simulink model "ASM_Traffic_new"  (R2024a)
settings: Solver=ode1  StartTime=SIM.tstart.v  StopTime=SIM.tend.v  FixedStep=SIM.StepSize.v  RelTol=1e-3
PostLoadFcn:
  | if any(exist('dsrtsu_mdlpostloadfcn', 'file') ~= 0), dsrtsu_mdlpostloadfcn('Execute', bdroot); end
  | try, asm_mdl_postloadfcn(bdroot, 'UpdateModel', 3600); catch, disp(lasterr); end,
InitFcn:
  | , if any(exist('rtifpga_mdlclblib', 'file') ~= 0), rtifpga_mdlclblib('Init', bdroot); end,
  | , if any(exist('dsmpb_private', 'file') ~= 0), dsmpb_private('dsmpb_mdlclblib', 'Init', bdroot); end,
undefined symbols (not defined in the file): _to_, a0b2, ASM_BrakeHydraulics_DemoSystems, ASM_VehicleDynamics_DemoSystems, b98103fe8ad365046cd0, BrakeCircuit, CPT, Crankshaft, DiscIntNeverNeededParam, dsmsi, FinalDriveAssembly, MDL, ModeSignals, Pos_BrakePedal_Maneuver, rad, RefSignals, s_to_rpm, SIM, SoftECU, Suspension, Tire, Transmission
libraries: ASM_Traffic_lib x135, simulink x100, ASM_Utils_lib x77, ASM_VehicleDynamics_lib x70, ASM_Environment_lib x22, dsmpblib x20, dsmsilib x15, MDLD_Utils_lib x10, ASM_BrakeHydraulics_lib x3
(part 24 of 63)

== system ASM_Traffic_new/Environment/Interface_Out/Animation/Mnv_Trunk[]_ ==
  In1 : Inport
  Gain : Gain  SaturateOnIntegerOverflow=on  OutDataTypeStr=Inherit: Same as input  ParamDataTypeStr=Inherit: Same as input
  Out1 : Outport  VectorParamsAs1DForOutWhenUnconnected=off
  wires:
  Gain/1 -> Out1/1
  In1/1 -> Gain/1

== system ASM_Traffic_new/Environment/Interface_Out/Animation/Network_Item_Type_Veh[]_ ==
  In1 : Inport
  Gain : Gain  SaturateOnIntegerOverflow=on  OutDataTypeStr=Inherit: Same as input  ParamDataTypeStr=Inherit: Same as input
  Out1 : Outport  VectorParamsAs1DForOutWhenUnconnected=off
  wires:
  Gain/1 -> Out1/1
  In1/1 -> Gain/1

== system ASM_Traffic_new/Environment/Interface_Out/Animation/Pos_Left[x;y;z][m]_ ==
  In1 : Inport
  Gain : Gain  SaturateOnIntegerOverflow=on  OutDataTypeStr=Inherit: Same as input  ParamDataTypeStr=Inherit: Same as input
  Out1 : Outport  VectorParamsAs1DForOutWhenUnconnected=off
  wires:
  Gain/1 -> Out1/1
  In1/1 -> Gain/1

== system ASM_Traffic_new/Environment/Interface_Out/Animation/Pos_Right[x;y;z][m]_ ==
  In1 : Inport
  Gain : Gain  SaturateOnIntegerOverflow=on  OutDataTypeStr=Inherit: Same as input  ParamDataTypeStr=Inherit: Same as input
  Out1 : Outport  VectorParamsAs1DForOutWhenUnconnected=off
  wires:
  In1/1 -> Gain/1
  Gain/1 -> Out1/1

== system ASM_Traffic_new/Environment/Interface_Out/Animation/Sw_AnimationInterface[0Disabled|1Enabled]_ ==
  In1 : Inport
  Gain : Gain  SaturateOnIntegerOverflow=on  OutDataTypeStr=Inherit: Same as input  ParamDataTypeStr=Inherit: Same as input
  Out1 : Outport  VectorParamsAs1DForOutWhenUnconnected=off
  wires:
  Gain/1 -> Out1/1
  In1/1 -> Gain/1

== system ASM_Traffic_new/Environment/Interface_Out/Animation/Sw_BrakeLight[0Off|1On]_ ==
  In1 : Inport
  Gain : Gain  SaturateOnIntegerOverflow=on  OutDataTypeStr=Inherit: Same as input  ParamDataTypeStr=Inherit: Same as input
  Out1 : Outport  VectorParamsAs1DForOutWhenUnconnected=off
  wires:
  Gain/1 -> Out1/1
  In1/1 -> Gain/1

== system ASM_Traffic_new/Environment/Interface_Out/Animation/Sw_DoorFL[0Closed_1Open]_ ==
  In1 : Inport
  Gain : Gain  SaturateOnIntegerOverflow=on  OutDataTypeStr=Inherit: Same as input  ParamDataTypeStr=Inherit: Same as input
  Out1 : Outport  VectorParamsAs1DForOutWhenUnconnected=off
  wires:
  Gain/1 -> Out1/1
  In1/1 -> Gain/1

== system ASM_Traffic_new/Environment/Interface_Out/Animation/Sw_DoorFR[0Closed_1Open]_ ==
  In1 : Inport
  Gain : Gain  SaturateOnIntegerOverflow=on  OutDataTypeStr=Inherit: Same as input  ParamDataTypeStr=Inherit: Same as input
  Out1 : Outport  VectorParamsAs1DForOutWhenUnconnected=off
  wires:
  Gain/1 -> Out1/1
  In1/1 -> Gain/1

== system ASM_Traffic_new/Environment/Interface_Out/Animation/Sw_DoorRL[0Closed_1Open]_ ==
  In1 : Inport
  Gain : Gain  SaturateOnIntegerOverflow=on  OutDataTypeStr=Inherit: Same as input  ParamDataTypeStr=Inherit: Same as input
  Out1 : Outport  VectorParamsAs1DForOutWhenUnconnected=off
  wires:
  Gain/1 -> Out1/1
  In1/1 -> Gain/1

== system ASM_Traffic_new/Environment/Interface_Out/Animation/Sw_DoorRR[0Closed_1Open]_ ==
  In1 : Inport
  Gain : Gain  SaturateOnIntegerOverflow=on  OutDataTypeStr=Inherit: Same as input  ParamDataTypeStr=Inherit: Same as input
  Out1 : Outport  VectorParamsAs1DForOutWhenUnconnected=off
  wires:
  In1/1 -> Gain/1
  Gain/1 -> Out1/1

== system ASM_Traffic_new/Environment/Interface_Out/Animation/Sw_Hood[0Closed_1Open]_ ==
  In1 : Inport
  Gain : Gain  SaturateOnIntegerOverflow=on  OutDataTypeStr=Inherit: Same as input  ParamDataTypeStr=Inherit: Same as input
  Out1 : Outport  VectorParamsAs1DForOutWhenUnconnected=off
  wires:
  Gain/1 -> Out1/1
  In1/1 -> Gain/1

== system ASM_Traffic_new/Environment/Interface_Out/Animation/Sw_ManualControl_Doors[1Maneuver|2Manual]_ ==
  In1 : Inport
  Gain : Gain  SaturateOnIntegerOverflow=on  OutDataTypeStr=Inherit: Same as input  ParamDataTypeStr=Inherit: Same as input
  Out1 : Outport  VectorParamsAs1DForOutWhenUnconnected=off
  wires:
  Gain/1 -> Out1/1
  In1/1 -> Gain/1

== system ASM_Traffic_new/Environment/Interface_Out/Animation/Sw_ManualControl_Lights[1Maneuver|2Manual]_ ==
  In1 : Inport
  Gain : Gain  SaturateOnIntegerOverflow=on  OutDataTypeStr=Inherit: Same as input  ParamDataTypeStr=Inherit: Same as input
  Out1 : Outport  VectorParamsAs1DForOutWhenUnconnected=off
  wires:
  In1/1 -> Gain/1
  Gain/1 -> Out1/1

== system ASM_Traffic_new/Environment/Interface_Out/Animation/Sw_Trunk[0Closed_1Open]_ ==
  In1 : Inport
  Gain : Gain  SaturateOnIntegerOverflow=on  OutDataTypeStr=Inherit: Same as input  ParamDataTypeStr=Inherit: Same as input
  Out1 : Outport  VectorParamsAs1DForOutWhenUnconnected=off
  wires:
  In1/1 -> Gain/1
  Gain/1 -> Out1/1

== system ASM_Traffic_new/Environment/Interface_Out/Animation/Sw_TurnLights[0Off|1Left|2Right|3Both]_ ==
  In1 : Inport
  Gain : Gain  SaturateOnIntegerOverflow=on  OutDataTypeStr=Inherit: Same as input  ParamDataTypeStr=Inherit: Same as input
  Out1 : Outport  VectorParamsAs1DForOutWhenUnconnected=off
  wires:
  In1/1 -> Gain/1
  Gain/1 -> Out1/1

== system ASM_Traffic_new/Environment/Interface_Out/Animation/Velocity_MeasPnt_Marker_Left[m|s]_ ==
  In1 : Inport
  Gain : Gain  SaturateOnIntegerOverflow=on  OutDataTypeStr=Inherit: Same as input  ParamDataTypeStr=Inherit: Same as input
  Out1 : Outport  VectorParamsAs1DForOutWhenUnconnected=off
  wires:
  In1/1 -> Gain/1
  Gain/1 -> Out1/1

== system ASM_Traffic_new/Environment/Interface_Out/Animation/Velocity_MeasPnt_Marker_Right[m|s]_ ==
  In1 : Inport
  Gain : Gain  SaturateOnIntegerOverflow=on  OutDataTypeStr=Inherit: Same as input  ParamDataTypeStr=Inherit: Same as input
  Out1 : Outport  VectorParamsAs1DForOutWhenUnconnected=off
  wires:
  Gain/1 -> Out1/1
  In1/1 -> Gain/1

== system ASM_Traffic_new/Environment/Interface_Out/Animation/Yaw_Angle_Left[deg]_ ==
  In1 : Inport
  Gain : Gain  SaturateOnIntegerOverflow=on  OutDataTypeStr=Inherit: Same as input  ParamDataTypeStr=Inherit: Same as input
  Out1 : Outport  VectorParamsAs1DForOutWhenUnconnected=off
  wires:
  In1/1 -> Gain/1
  Gain/1 -> Out1/1

== system ASM_Traffic_new/Environment/Interface_Out/Animation/Yaw_Angle_Right[deg]_ ==
  In1 : Inport
  Gain : Gain  SaturateOnIntegerOverflow=on  OutDataTypeStr=Inherit: Same as input  ParamDataTypeStr=Inherit: Same as input
  Out1 : Outport  VectorParamsAs1DForOutWhenUnconnected=off
  wires:
  Gain/1 -> Out1/1
  In1/1 -> Gain/1

== system ASM_Traffic_new/Environment/Interface_Out/Animation/a_Fellows[m|s2] ==
  In1 : Inport
  Gain : Gain  SaturateOnIntegerOverflow=on  OutDataTypeStr=Inherit: Same as input  ParamDataTypeStr=Inherit: Same as input
  Out1 : Outport  VectorParamsAs1DForOutWhenUnconnected=off
  wires:
  Gain/1 -> Out1/1
  In1/1 -> Gain/1

== system ASM_Traffic_new/Environment/Interface_Out/Animation/s_Veh_Road[m]_ ==
  In1 : Inport
  Gain : Gain  SaturateOnIntegerOverflow=on  OutDataTypeStr=Inherit: Same as input  ParamDataTypeStr=Inherit: Same as input
  Out1 : Outport  VectorParamsAs1DForOutWhenUnconnected=off
  wires:
  In1/1 -> Gain/1
  Gain/1 -> Out1/1

== system ASM_Traffic_new/Environment/Interface_Out/Animation/v_Fellows[km|h]_ ==
  In1 : Inport
  Gain : Gain  SaturateOnIntegerOverflow=on  OutDataTypeStr=Inherit: Same as input  ParamDataTypeStr=Inherit: Same as input
  Out1 : Outport  VectorParamsAs1DForOutWhenUnconnected=off
  wires:
  In1/1 -> Gain/1
  Gain/1 -> Out1/1

== system ASM_Traffic_new/Environment/Interface_Out/Animation/v_Fellows_Ref_Scheduler[km|h]_ ==
  In1 : Inport
  Gain : Gain  SaturateOnIntegerOverflow=on  OutDataTypeStr=Inherit: Same as input  ParamDataTypeStr=Inherit: Same as input
  Out1 : Outport  VectorParamsAs1DForOutWhenUnconnected=off
  wires:
  Gain/1 -> Out1/1
  In1/1 -> Gain/1

== system ASM_Traffic_new/Environment/Interface_Out/Plant_ModelSignals/Activate_DCLink[0Off|1On]_ ==
  In1 : Inport
  Gain : Gain  SaturateOnIntegerOverflow=on  OutDataTypeStr=Inherit: Same as input  ParamDataTypeStr=Inherit: Same as input
  Out1 : Outport  VectorParamsAs1DForOutWhenUnconnected=off
  wires:
  In1/1 -> Gain/1
  Gain/1 -> Out1/1

== system ASM_Traffic_new/Environment/Interface_Out/Plant_ModelSignals/Angle_Hor_Rel_Fellows[deg]_ ==
  In1 : Inport
  Gain : Gain  SaturateOnIntegerOverflow=on  OutDataTypeStr=Inherit: Same as input  ParamDataTypeStr=Inherit: Same as input
  Out1 : Outport  VectorParamsAs1DForOutWhenUnconnected=off
  wires:
  In1/1 -> Gain/1
  Gain/1 -> Out1/1

== system ASM_Traffic_new/Environment/Interface_Out/Plant_ModelSignals/Angle_SteeringWheel_Maneuver[deg]_ ==
  In1 : Inport
  DummyGain : Gain  SaturateOnIntegerOverflow=on  OutDataTypeStr=Inherit: Same as input  ParamDataTypeStr=Inherit: Same as input
  Out1 : Outport  VectorParamsAs1DForOutWhenUnconnected=off
  wires:
  DummyGain/1 -> Out1/1
  In1/1 -> DummyGain/1

== system ASM_Traffic_new/Environment/Interface_Out/Plant_ModelSignals/Angle_Vehicle_Init_CoorSys_E[x;y;z][rad]_ ==
  In1 : Inport
  Gain : Gain  SaturateOnIntegerOverflow=on  OutDataTypeStr=Inherit: Same as input  ParamDataTypeStr=Inherit: Same as input
  Out1 : Outport  VectorParamsAs1DForOutWhenUnconnected=off
  wires:
  In1/1 -> Gain/1
  Gain/1 -> Out1/1

== system ASM_Traffic_new/Environment/Interface_Out/Plant_ModelSignals/Angle_Yaw_Veh_Road[deg]_ ==
  In1 : Inport
  Gain : Gain  SaturateOnIntegerOverflow=on  OutDataTypeStr=Inherit: Same as input  ParamDataTypeStr=Inherit: Same as input
  Out1 : Outport  VectorParamsAs1DForOutWhenUnconnected=off
  wires:
  In1/1 -> Gain/1
  Gain/1 -> Out1/1

== system ASM_Traffic_new/Environment/Interface_Out/Plant_ModelSignals/Const_Steering_Mode_Manual[1Angle|2Trq]_ ==
  In1 : Inport
  Gain : Gain  SaturateOnIntegerOverflow=on  OutDataTypeStr=Inherit: Same as input  ParamDataTypeStr=Inherit: Same as input
  Out1 : Outport  VectorParamsAs1DForOutWhenUnconnected=off
  wires:
  In1/1 -> Gain/1
  Gain/1 -> Out1/1

== system ASM_Traffic_new/Environment/Interface_Out/Plant_ModelSignals/Curv_Preview_Road[1|m]_ ==
  In1 : Inport
  Gain : Gain  SaturateOnIntegerOverflow=on  OutDataTypeStr=Inherit: Same as input  ParamDataTypeStr=Inherit: Same as input
  Out1 : Outport  VectorParamsAs1DForOutWhenUnconnected=off
  wires:
  Gain/1 -> Out1/1
  In1/1 -> Gain/1

== system ASM_Traffic_new/Environment/Interface_Out/Plant_ModelSignals/Curv_Vehicle_Road[1|m]_ ==
  In1 : Inport
  Gain : Gain  SaturateOnIntegerOverflow=on  OutDataTypeStr=Inherit: Same as input  ParamDataTypeStr=Inherit: Same as input
  Out1 : Outport  VectorParamsAs1DForOutWhenUnconnected=off
  wires:
  Gain/1 -> Out1/1
  In1/1 -> Gain/1

== system ASM_Traffic_new/Environment/Interface_Out/Plant_ModelSignals/Dist_Border_Left[m]_ ==
  In1 : Inport
  Gain : Gain  SaturateOnIntegerOverflow=on  OutDataTypeStr=Inherit: Same as input  ParamDataTypeStr=Inherit: Same as input
  Out1 : Outport  VectorParamsAs1DForOutWhenUnconnected=off
  wires:
  Gain/1 -> Out1/1
  In1/1 -> Gain/1

== system ASM_Traffic_new/Environment/Interface_Out/Plant_ModelSignals/Dist_Border_Right[m]_ ==
  In1 : Inport
  Gain : Gain  SaturateOnIntegerOverflow=on  OutDataTypeStr=Inherit: Same as input  ParamDataTypeStr=Inherit: Same as input
  Out1 : Outport  VectorParamsAs1DForOutWhenUnconnected=off
  wires:
  In1/1 -> Gain/1
  Gain/1 -> Out1/1

== system ASM_Traffic_new/Environment/Interface_Out/Plant_ModelSignals/Dist_Fellows[m]_ ==
  In1 : Inport
  Gain : Gain  SaturateOnIntegerOverflow=on  OutDataTypeStr=Inherit: Same as input  ParamDataTypeStr=Inherit: Same as input
  Out1 : Outport  VectorParamsAs1DForOutWhenUnconnected=off
  wires:
  In1/1 -> Gain/1
  Gain/1 -> Out1/1

== system ASM_Traffic_new/Environment/Interface_Out/Plant_ModelSignals/ECU_Commands[]_ ==
  In1 : Inport
  Gain : Gain  SaturateOnIntegerOverflow=on  OutDataTypeStr=Inherit: Same as input  ParamDataTypeStr=Inherit: Same as input
  Out1 : Outport  VectorParamsAs1DForOutWhenUnconnected=off
  wires:
  In1/1 -> Gain/1
  Gain/1 -> Out1/1

== system ASM_Traffic_new/Environment/Interface_Out/Plant_ModelSignals/Enable_v_Init[0|1]_ ==
  In1 : Inport
  DummyGain : Gain  SaturateOnIntegerOverflow=on  OutDataTypeStr=Inherit: Same as input  ParamDataTypeStr=Inherit: Same as input
  Out1 : Outport  VectorParamsAs1DForOutWhenUnconnected=off
  wires:
  DummyGain/1 -> Out1/1
  In1/1 -> DummyGain/1

== system ASM_Traffic_new/Environment/Interface_Out/Plant_ModelSignals/EngOPNum[]_ ==
  In1 : Inport
  DummyGain : Gain  SaturateOnIntegerOverflow=on  OutDataTypeStr=Inherit: Same as input  ParamDataTypeStr=Inherit: Same as input
  Out1 : Outport  VectorParamsAs1DForOutWhenUnconnected=off
  wires:
  DummyGain/1 -> Out1/1
  In1/1 -> DummyGain/1

== system ASM_Traffic_new/Environment/Interface_Out/Plant_ModelSignals/Fric_Coeff_CP[:][]_ ==
  In1 : Inport
  Gain : Gain  SaturateOnIntegerOverflow=on  OutDataTypeStr=Inherit: Same as input  ParamDataTypeStr=Inherit: Same as input
  Out1 : Outport  VectorParamsAs1DForOutWhenUnconnected=off
  wires:
  In1/1 -> Gain/1
  Gain/1 -> Out1/1

== system ASM_Traffic_new/Environment/Interface_Out/Plant_ModelSignals/Gear_Maneuver[]_ ==
  In1 : Inport
  DummyGain : Gain  SaturateOnIntegerOverflow=on  OutDataTypeStr=Inherit: Same as input  ParamDataTypeStr=Inherit: Same as input
  Out1 : Outport  VectorParamsAs1DForOutWhenUnconnected=off
  wires:
  In1/1 -> DummyGain/1
  DummyGain/1 -> Out1/1

== system ASM_Traffic_new/Environment/Interface_Out/Plant_ModelSignals/Gear_Max[0Off|1_n]_ ==
  In1 : Inport
  DummyGain : Gain  SaturateOnIntegerOverflow=on  OutDataTypeStr=Inherit: Same as input  ParamDataTypeStr=Inherit: Same as input
  Out1 : Outport  VectorParamsAs1DForOutWhenUnconnected=off
  wires:
  In1/1 -> DummyGain/1
  DummyGain/1 -> Out1/1

== system ASM_Traffic_new/Environment/Interface_Out/Plant_ModelSignals/Height_Fellows[m]_ ==
  In1 : Inport
  Gain : Gain  SaturateOnIntegerOverflow=on  OutDataTypeStr=Inherit: Same as input  ParamDataTypeStr=Inherit: Same as input
  Out1 : Outport  VectorParamsAs1DForOutWhenUnconnected=off
  wires:
  In1/1 -> Gain/1
  Gain/1 -> Out1/1

== system ASM_Traffic_new/Environment/Interface_Out/Plant_ModelSignals/I_Load_HV[A]_ ==
  In1 : Inport
  Gain : Gain  SaturateOnIntegerOverflow=on  OutDataTypeStr=Inherit: Same as input  ParamDataTypeStr=Inherit: Same as input
  Out1 : Outport  VectorParamsAs1DForOutWhenUnconnected=off
  wires:
  Gain/1 -> Out1/1
  In1/1 -> Gain/1

== system ASM_Traffic_new/Environment/Interface_Out/Plant_ModelSignals/I_Load_LV[A]_ ==
  In1 : Inport
  Gain : Gain  SaturateOnIntegerOverflow=on  OutDataTypeStr=Inherit: Same as input  ParamDataTypeStr=Inherit: Same as input
  Out1 : Outport  VectorParamsAs1DForOutWhenUnconnected=off
  wires:
  In1/1 -> Gain/1
  Gain/1 -> Out1/1

== system ASM_Traffic_new/Environment/Interface_Out/Plant_ModelSignals/Keep_VehiclePosition[0|1]_ ==
  In1 : Inport
  Gain : Gain  SaturateOnIntegerOverflow=on  OutDataTypeStr=Inherit: Same as input  ParamDataTypeStr=Inherit: Same as input
  Out1 : Outport  VectorParamsAs1DForOutWhenUnconnected=off
  wires:
  In1/1 -> Gain/1
  Gain/1 -> Out1/1

== system ASM_Traffic_new/Environment/Interface_Out/Plant_ModelSignals/Lane_ID_Vehicle[]_ ==
  In1 : Inport
  Gain : Gain  SaturateOnIntegerOverflow=on  OutDataTypeStr=Inherit: Same as input  ParamDataTypeStr=Inherit: Same as input
  Out1 : Outport  VectorParamsAs1DForOutWhenUnconnected=off
  wires:
  In1/1 -> Gain/1
  Gain/1 -> Out1/1

== system ASM_Traffic_new/Environment/Interface_Out/Plant_ModelSignals/Length_Fellows[m]_ ==
  In1 : Inport
  Gain : Gain  SaturateOnIntegerOverflow=on  OutDataTypeStr=Inherit: Same as input  ParamDataTypeStr=Inherit: Same as input
  Out1 : Outport  VectorParamsAs1DForOutWhenUnconnected=off
  wires:
  In1/1 -> Gain/1
  Gain/1 -> Out1/1

== system ASM_Traffic_new/Environment/Interface_Out/Plant_ModelSignals/Mode_AcceleratorBrake[1Stim|2Driver]_ ==
  In1 : Inport
  Gain : Gain  SaturateOnIntegerOverflow=on  OutDataTypeStr=Inherit: Same as input  ParamDataTypeStr=Inherit: Same as input
  Out1 : Outport  VectorParamsAs1DForOutWhenUnconnected=off
  wires:
  In1/1 -> Gain/1
  Gain/1 -> Out1/1

== system ASM_Traffic_new/Environment/Interface_Out/Plant_ModelSignals/Mode_AdaptVelocityToRoad[1Off|2On]_ ==
  In1 : Inport
  Gain : Gain  SaturateOnIntegerOverflow=on  OutDataTypeStr=Inherit: Same as input  ParamDataTypeStr=Inherit: Same as input
  Out1 : Outport  VectorParamsAs1DForOutWhenUnconnected=off
  wires:
  In1/1 -> Gain/1
  Gain/1 -> Out1/1

== system ASM_Traffic_new/Environment/Interface_Out/Plant_ModelSignals/Mode_CurvatureCalculation[1Road|2Driver]_ ==
  In1 : Inport
  Gain : Gain  SaturateOnIntegerOverflow=on  OutDataTypeStr=Inherit: Same as input  ParamDataTypeStr=Inherit: Same as input
  Out1 : Outport  VectorParamsAs1DForOutWhenUnconnected=off
  wires:
  In1/1 -> Gain/1
  Gain/1 -> Out1/1

== system ASM_Traffic_new/Environment/Interface_Out/Plant_ModelSignals/Mode_ForceToRoad[1Off|2On]_ ==
  In1 : Inport
  Gain : Gain  SaturateOnIntegerOverflow=on  OutDataTypeStr=Inherit: Same as input  ParamDataTypeStr=Inherit: Same as input
  Out1 : Outport  VectorParamsAs1DForOutWhenUnconnected=off
  wires:
  Gain/1 -> Out1/1
  In1/1 -> Gain/1

== system ASM_Traffic_new/Environment/Interface_Out/Plant_ModelSignals/Mode_GearClutch[1Stim|2Driver|3OpenClutch|4RefGear]_ ==
  In1 : Inport
  Gain : Gain  SaturateOnIntegerOverflow=on  OutDataTypeStr=Inherit: Same as input  ParamDataTypeStr=Inherit: Same as input
  Out1 : Outport  VectorParamsAs1DForOutWhenUnconnected=off
  wires:
  Gain/1 -> Out1/1
  In1/1 -> Gain/1

== system ASM_Traffic_new/Environment/Interface_Out/Plant_ModelSignals/Mode_LatCtrl[1Pos|2Yaw]_ ==
  In1 : Inport
  Gain : Gain  SaturateOnIntegerOverflow=on  OutDataTypeStr=Inherit: Same as input  ParamDataTypeStr=Inherit: Same as input
  Out1 : Outport  VectorParamsAs1DForOutWhenUnconnected=off
  wires:
  Gain/1 -> Out1/1
  In1/1 -> Gain/1

== system ASM_Traffic_new/Environment/Interface_Out/Plant_ModelSignals/Mode_RelativeLane[0CenterLane|1PreferredLane]_ ==
  In1 : Inport
  Gain : Gain  SaturateOnIntegerOverflow=on  OutDataTypeStr=Inherit: Same as input  ParamDataTypeStr=Inherit: Same as input
  Out1 : Outport  VectorParamsAs1DForOutWhenUnconnected=off
  wires:
  In1/1 -> Gain/1
  Gain/1 -> Out1/1

== system ASM_Traffic_new/Environment/Interface_Out/Plant_ModelSignals/Mode_Road[1NoRoad|2Straight|3Circle|4Road]_ ==
  In1 : Inport
  Gain : Gain  SaturateOnIntegerOverflow=on  OutDataTypeStr=Inherit: Same as input  ParamDataTypeStr=Inherit: Same as input
  Out1 : Outport  VectorParamsAs1DForOutWhenUnconnected=off
  wires:
  Gain/1 -> Out1/1
  In1/1 -> Gain/1

== system ASM_Traffic_new/Environment/Interface_Out/Plant_ModelSignals/Mode_SelectorLever[1Stim|2Driver]_ ==
  In1 : Inport
  Gain : Gain  SaturateOnIntegerOverflow=on  OutDataTypeStr=Inherit: Same as input  ParamDataTypeStr=Inherit: Same as input
  Out1 : Outport  VectorParamsAs1DForOutWhenUnconnected=off
  wires:
  In1/1 -> Gain/1
  Gain/1 -> Out1/1

== system ASM_Traffic_new/Environment/Interface_Out/Plant_ModelSignals/Mode_StartButtonState[1Stim|2SoftECU]_ ==
  In1 : Inport
  Gain : Gain  SaturateOnIntegerOverflow=on  OutDataTypeStr=Inherit: Same as input  ParamDataTypeStr=Inherit: Same as input
  Out1 : Outport  VectorParamsAs1DForOutWhenUnconnected=off
  wires:
  Gain/1 -> Out1/1
  In1/1 -> Gain/1

== system ASM_Traffic_new/Environment/Interface_Out/Plant_ModelSignals/Mode_Steer[1Stim|2Driver|3Fix]_ ==
  In1 : Inport
  Gain : Gain  SaturateOnIntegerOverflow=on  OutDataTypeStr=Inherit: Same as input  ParamDataTypeStr=Inherit: Same as input
  Out1 : Outport  VectorParamsAs1DForOutWhenUnconnected=off
  wires:
  In1/1 -> Gain/1
  Gain/1 -> Out1/1

== system ASM_Traffic_new/Environment/Interface_Out/Plant_ModelSignals/Mode_TrafficDriver[1Off|2On]_ ==
  In1 : Inport
  Gain : Gain  SaturateOnIntegerOverflow=on  OutDataTypeStr=Inherit: Same as input  ParamDataTypeStr=Inherit: Same as input
  Out1 : Outport  VectorParamsAs1DForOutWhenUnconnected=off
  wires:
  Gain/1 -> Out1/1
  In1/1 -> Gain/1

== system ASM_Traffic_new/Environment/Interface_Out/Plant_ModelSignals/Object_ID[]_ ==
  In1 : Inport
  Gain : Gain  SaturateOnIntegerOverflow=on  OutDataTypeStr=Inherit: Same as input  ParamDataTypeStr=Inherit: Same as input
  Out1 : Outport  VectorParamsAs1DForOutWhenUnconnected=off
  wires:
  In1/1 -> Gain/1
  Gain/1 -> Out1/1

== system ASM_Traffic_new/Environment/Interface_Out/Plant_ModelSignals/Pitch_Preview_Road[deg]_ ==
  In1 : Inport
  Gain : Gain  SaturateOnIntegerOverflow=on  OutDataTypeStr=Inherit: Same as input  ParamDataTypeStr=Inherit: Same as input
  Out1 : Outport  VectorParamsAs1DForOutWhenUnconnected=off
  wires:
  Gain/1 -> Out1/1
  In1/1 -> Gain/1

== system ASM_Traffic_new/Environment/Interface_Out/Plant_ModelSignals/PosVec_MainPnt_Fellows[x;y;z][m]_ ==
  In1 : Inport
  Gain : Gain  SaturateOnIntegerOverflow=on  OutDataTypeStr=Inherit: Same as input  ParamDataTypeStr=Inherit: Same as input
  Out1 : Outport  VectorParamsAs1DForOutWhenUnconnected=off
  wires:
  In1/1 -> Gain/1
  Gain/1 -> Out1/1

== system ASM_Traffic_new/Environment/Interface_Out/Plant_ModelSignals/Pos_AccPedal_Maneuver[%]_ ==
  In1 : Inport
  DummyGain : Gain  SaturateOnIntegerOverflow=on  OutDataTypeStr=Inherit: Same as input  ParamDataTypeStr=Inherit: Same as input
  Out1 : Outport  VectorParamsAs1DForOutWhenUnconnected=off
  wires:
  In1/1 -> DummyGain/1
  DummyGain/1 -> Out1/1

== system ASM_Traffic_new/Environment/Interface_Out/Plant_ModelSignals/Pos_BrakePedal_Maneuver[%]_ ==
  In1 : Inport
  DummyGain : Gain  SaturateOnIntegerOverflow=on  OutDataTypeStr=Inherit: Same as input  ParamDataTypeStr=Inherit: Same as input
  Out1 : Outport  VectorParamsAs1DForOutWhenUnconnected=off
  wires:
  In1/1 -> DummyGain/1
  DummyGain/1 -> Out1/1

== system ASM_Traffic_new/Environment/Interface_Out/Plant_ModelSignals/Pos_ClutchPedal_Maneuver[%]_ ==
  In1 : Inport
  DummyGain : Gain  SaturateOnIntegerOverflow=on  OutDataTypeStr=Inherit: Same as input  ParamDataTypeStr=Inherit: Same as input
  Out1 : Outport  VectorParamsAs1DForOutWhenUnconnected=off
  wires:
  In1/1 -> DummyGain/1
  DummyGain/1 -> Out1/1

== system ASM_Traffic_new/Environment/Interface_Out/Plant_ModelSignals/Pos_Vehicle_Init_CoorSys_E[x;y;z][m]_ ==
  In1 : Inport
  Gain : Gain  SaturateOnIntegerOverflow=on  OutDataTypeStr=Inherit: Same as input  ParamDataTypeStr=Inherit: Same as input
  Out1 : Outport  VectorParamsAs1DForOutWhenUnconnected=off
  wires:
  In1/1 -> Gain/1
  Gain/1 -> Out1/1

== system ASM_Traffic_new/Environment/Interface_Out/Plant_ModelSignals/Pos_x_Preview_Road[m]_ ==
  In1 : Inport
  Gain : Gain  SaturateOnIntegerOverflow=on  OutDataTypeStr=Inherit: Same as input  ParamDataTypeStr=Inherit: Same as input
  Out1 : Outport  VectorParamsAs1DForOutWhenUnconnected=off
  wires:
  Gain/1 -> Out1/1
  In1/1 -> Gain/1

== system ASM_Traffic_new/Environment/Interface_Out/Plant_ModelSignals/Pos_x_Ref_Vehicle_Road[m]_ ==
  In1 : Inport
  Gain : Gain  SaturateOnIntegerOverflow=on  OutDataTypeStr=Inherit: Same as input  ParamDataTypeStr=Inherit: Same as input
  Out1 : Outport  VectorParamsAs1DForOutWhenUnconnected=off
  wires:
  Gain/1 -> Out1/1
  In1/1 -> Gain/1

== system ASM_Traffic_new/Environment/Interface_Out/Plant_ModelSignals/Pos_y_Preview_Road[m]_ ==
  In1 : Inport
  Gain : Gain  SaturateOnIntegerOverflow=on  OutDataTypeStr=Inherit: Same as input  ParamDataTypeStr=Inherit: Same as input
  Out1 : Outport  VectorParamsAs1DForOutWhenUnconnected=off
  wires:
  In1/1 -> Gain/1
  Gain/1 -> Out1/1

== system ASM_Traffic_new/Environment/Interface_Out/Plant_ModelSignals/Pos_y_Ref_Vehicle_Road[m]_ ==
  In1 : Inport
  Gain : Gain  SaturateOnIntegerOverflow=on  OutDataTypeStr=Inherit: Same as input  ParamDataTypeStr=Inherit: Same as input
  Out1 : Outport  VectorParamsAs1DForOutWhenUnconnected=off
  wires:
  In1/1 -> Gain/1
  Gain/1 -> Out1/1

== system ASM_Traffic_new/Environment/Interface_Out/Plant_ModelSignals/Pos_z_CP[:][m]_ ==
  In1 : Inport
  Gain : Gain  SaturateOnIntegerOverflow=on  OutDataTypeStr=Inherit: Same as input  ParamDataTypeStr=Inherit: Same as input
  Out1 : Outport  VectorParamsAs1DForOutWhenUnconnected=off
  wires:
  In1/1 -> Gain/1
  Gain/1 -> Out1/1

== system ASM_Traffic_new/Environment/Interface_Out/Plant_ModelSignals/Pos_z_Preview_Road[m]_ ==
  In1 : Inport
  Gain : Gain  SaturateOnIntegerOverflow=on  OutDataTypeStr=Inherit: Same as input  ParamDataTypeStr=Inherit: Same as input
  Out1 : Outport  VectorParamsAs1DForOutWhenUnconnected=off
  wires:
  Gain/1 -> Out1/1
  In1/1 -> Gain/1

== system ASM_Traffic_new/Environment/Interface_Out/Plant_ModelSignals/Reset_VehicleStates[0|1]_ ==
  In1 : Inport
  Gain : Gain  SaturateOnIntegerOverflow=on  OutDataTypeStr=Inherit: Same as input  ParamDataTypeStr=Inherit: Same as input
  Out1 : Outport  VectorParamsAs1DForOutWhenUnconnected=off
  wires:
  In1/1 -> Gain/1
  Gain/1 -> Out1/1

== system ASM_Traffic_new/Environment/Interface_Out/Plant_ModelSignals/Roll_Preview_Road[deg]_ ==
  In1 : Inport
  Gain : Gain  SaturateOnIntegerOverflow=on  OutDataTypeStr=Inherit: Same as input  ParamDataTypeStr=Inherit: Same as input
  Out1 : Outport  VectorParamsAs1DForOutWhenUnconnected=off
  wires:
  In1/1 -> Gain/1
  Gain/1 -> Out1/1

== system ASM_Traffic_new/Environment/Interface_Out/Plant_ModelSignals/Route_Direction_Init[]_ ==
  In1 : Inport
  Gain : Gain  SaturateOnIntegerOverflow=on  OutDataTypeStr=Inherit: Same as input  ParamDataTypeStr=Inherit: Same as input
  Out1 : Outport  VectorParamsAs1DForOutWhenUnconnected=off
  wires:
  Gain/1 -> Out1/1
  In1/1 -> Gain/1

== system ASM_Traffic_new/Environment/Interface_Out/Plant_ModelSignals/SelectorLever_Maneuver[-3T|-2P|-1R|0N|1D]_ ==
  In1 : Inport
  DummyGain : Gain  SaturateOnIntegerOverflow=on  OutDataTypeStr=Inherit: Same as input  ParamDataTypeStr=Inherit: Same as input
  Out1 : Outport  VectorParamsAs1DForOutWhenUnconnected=off
  wires:
  In1/1 -> DummyGain/1
  DummyGain/1 -> Out1/1

== system ASM_Traffic_new/Environment/Interface_Out/Plant_ModelSignals/Slope_Veh_Road[%]_ ==
  In1 : Inport
  Gain : Gain  SaturateOnIntegerOverflow=on  OutDataTypeStr=Inherit: Same as input  ParamDataTypeStr=Inherit: Same as input
  Out1 : Outport  VectorParamsAs1DForOutWhenUnconnected=off
  wires:
  In1/1 -> Gain/1
  Gain/1 -> Out1/1

== system ASM_Traffic_new/Environment/Interface_Out/Plant_ModelSignals/Speed_Limit_Preview_Road[km|h]_ ==
  In1 : Inport
  Gain : Gain  SaturateOnIntegerOverflow=on  OutDataTypeStr=Inherit: Same as input  ParamDataTypeStr=Inherit: Same as input
  Out1 : Outport  VectorParamsAs1DForOutWhenUnconnected=off
  wires:
  In1/1 -> Gain/1
  Gain/1 -> Out1/1

== system ASM_Traffic_new/Environment/Interface_Out/Plant_ModelSignals/State_StartButton[-1PowerOff|0Acc|1PowerOn|2StarterOn]_ ==
  In1 : Inport
  Gain : Gain  SaturateOnIntegerOverflow=on  OutDataTypeStr=Inherit: Same as input  ParamDataTypeStr=Inherit: Same as input
  Out1 : Outport  VectorParamsAs1DForOutWhenUnconnected=off
  wires:
  In1/1 -> Gain/1
  Gain/1 -> Out1/1

== system ASM_Traffic_new/Environment/Interface_Out/Plant_ModelSignals/Sw_LatDriver[1LatCtrl1|2LatCtrl2]_ ==
  In1 : Inport
  Gain : Gain  SaturateOnIntegerOverflow=on  OutDataTypeStr=Inherit: Same as input  ParamDataTypeStr=Inherit: Same as input
  Out1 : Outport  VectorParamsAs1DForOutWhenUnconnected=off
  wires:
  In1/1 -> Gain/1
  Gain/1 -> Out1/1

== system ASM_Traffic_new/Environment/Interface_Out/Plant_ModelSignals/Sw_ModelDeskPlottingInterface[0Disabled|1Enabled]_ ==
  In1 : Inport
  Gain : Gain  SaturateOnIntegerOverflow=on  OutDataTypeStr=Inherit: Same as input  ParamDataTypeStr=Inherit: Same as input
  Out1 : Outport  VectorParamsAs1DForOutWhenUnconnected=off
  wires:
  In1/1 -> Gain/1
  Gain/1 -> Out1/1

== system ASM_Traffic_new/Environment/Interface_Out/Plant_ModelSignals/Sw_ModelPortBlocks[0Disabled|1Enabled]_ ==
  In1 : Inport
  Gain : Gain  SaturateOnIntegerOverflow=on  OutDataTypeStr=Inherit: Same as input  ParamDataTypeStr=Inherit: Same as input
  Out1 : Outport  VectorParamsAs1DForOutWhenUnconnected=off
  wires:
  In1/1 -> Gain/1
  Gain/1 -> Out1/1

== system ASM_Traffic_new/Environment/Interface_Out/Plant_ModelSignals/Sw_ParkingBrake[0Off|1On]_ ==
  In1 : Inport
  Gain : Gain  SaturateOnIntegerOverflow=on  OutDataTypeStr=Inherit: Same as input  ParamDataTypeStr=Inherit: Same as input
  Out1 : Outport  VectorParamsAs1DForOutWhenUnconnected=off
  wires:
  In1/1 -> Gain/1
  Gain/1 -> Out1/1

== system ASM_Traffic_new/Environment/Interface_Out/Plant_ModelSignals/Sw_StartButton[0Off|1On]_ ==
  In1 : Inport
  DummyGain : Gain  SaturateOnIntegerOverflow=on  OutDataTypeStr=Inherit: Same as input  ParamDataTypeStr=Inherit: Same as input
  Out1 : Outport  VectorParamsAs1DForOutWhenUnconnected=off
  wires:
  In1/1 -> DummyGain/1
  DummyGain/1 -> Out1/1

== system ASM_Traffic_new/Environment/Interface_Out/Plant_ModelSignals/Sw_SteeringMode[1Angle|2Trq]_ ==
  In1 : Inport
  Gain : Gain  SaturateOnIntegerOverflow=on  OutDataTypeStr=Inherit: Same as input  ParamDataTypeStr=Inherit: Same as input
  Out1 : Outport  VectorParamsAs1DForOutWhenUnconnected=off
  wires:
  In1/1 -> Gain/1
  Gain/1 -> Out1/1

== system ASM_Traffic_new/Environment/Interface_Out/Plant_ModelSignals/Sw_Steering_Mode[1Manual|2ManSched]_ ==
  In1 : Inport
  Gain : Gain  SaturateOnIntegerOverflow=on  OutDataTypeStr=Inherit: Same as input  ParamDataTypeStr=Inherit: Same as input
  Out1 : Outport  VectorParamsAs1DForOutWhenUnconnected=off
  wires:
  Gain/1 -> Out1/1
  In1/1 -> Gain/1

== system ASM_Traffic_new/Environment/Interface_Out/Plant_ModelSignals/Sw_Testbench[0Off|1On]_ ==
  In1 : Inport
  Gain : Gain  SaturateOnIntegerOverflow=on  OutDataTypeStr=Inherit: Same as input  ParamDataTypeStr=Inherit: Same as input
  Out1 : Outport  VectorParamsAs1DForOutWhenUnconnected=off
  wires:
  In1/1 -> Gain/1
  Gain/1 -> Out1/1

== system ASM_Traffic_new/Environment/Interface_Out/Plant_ModelSignals/Sw_TipShift_Maneuver[-1Down|0Off|1Up]_ ==
  In1 : Inport
  DummyGain : Gain  SaturateOnIntegerOverflow=on  OutDataTypeStr=Inherit: Same as input  ParamDataTypeStr=Inherit: Same as input
  Out1 : Outport  VectorParamsAs1DForOutWhenUnconnected=off
  wires:
  In1/1 -> DummyGain/1
  DummyGain/1 -> Out1/1

== system ASM_Traffic_new/Environment/Interface_Out/Plant_ModelSignals/Sw_Tire_Parameter_Set_CP[:][1|2|3|4]_ ==
  In1 : Inport
  Gain : Gain  SaturateOnIntegerOverflow=on  OutDataTypeStr=Inherit: Same as input  ParamDataTypeStr=Inherit: Same as input
  Out1 : Outport  VectorParamsAs1DForOutWhenUnconnected=off
  wires:
  In1/1 -> Gain/1
  Gain/1 -> Out1/1

== system ASM_Traffic_new/Environment/Interface_Out/Plant_ModelSignals/T_Ambient[degC]_ ==
  In1 : Inport
  Gain : Gain  SaturateOnIntegerOverflow=on  OutDataTypeStr=Inherit: Same as input  ParamDataTypeStr=Inherit: Same as input
  Out1 : Outport  VectorParamsAs1DForOutWhenUnconnected=off
  wires:
  In1/1 -> Gain/1
  Gain/1 -> Out1/1

== system ASM_Traffic_new/Environment/Interface_Out/Plant_ModelSignals/Trq_Driver_External[Nm]_ ==
  In1 : Inport
  Gain : Gain  SaturateOnIntegerOverflow=on  OutDataTypeStr=Inherit: Same as input  ParamDataTypeStr=Inherit: Same as input
  Out1 : Outport  VectorParamsAs1DForOutWhenUnconnected=off
  wires:
  In1/1 -> Gain/1
  Gain/1 -> Out1/1

== system ASM_Traffic_new/Environment/Interface_Out/Plant_ModelSignals/UnitVec_z_CP[:][x;y;z]_ ==
  In1 : Inport
  Gain : Gain  SaturateOnIntegerOverflow=on  OutDataTypeStr=Inherit: Same as input  ParamDataTypeStr=Inherit: Same as input
  Out1 : Outport  VectorParamsAs1DForOutWhenUnconnected=off
  wires:
  In1/1 -> Gain/1
  Gain/1 -> Out1/1

== system ASM_Traffic_new/Environment/Interface_Out/Plant_ModelSignals/Width_Deadzone_LatCtrl[m]_ ==
  In1 : Inport
  Gain : Gain  SaturateOnIntegerOverflow=on  OutDataTypeStr=Inherit: Same as input  ParamDataTypeStr=Inherit: Same as input
  Out1 : Outport  VectorParamsAs1DForOutWhenUnconnected=off
  wires:
  In1/1 -> Gain/1
  Gain/1 -> Out1/1

== system ASM_Traffic_new/Environment/Interface_Out/Plant_ModelSignals/Width_Fellows[m]_ ==
  In1 : Inport
  Gain : Gain  SaturateOnIntegerOverflow=on  OutDataTypeStr=Inherit: Same as input  ParamDataTypeStr=Inherit: Same as input
  Out1 : Outport  VectorParamsAs1DForOutWhenUnconnected=off
  wires:
  In1/1 -> Gain/1
  Gain/1 -> Out1/1

== system ASM_Traffic_new/Environment/Interface_Out/Plant_ModelSignals/a_x_Max[m|s2]_ ==
  In1 : Inport
  DummyGain : Gain  SaturateOnIntegerOverflow=on  OutDataTypeStr=Inherit: Same as input  ParamDataTypeStr=Inherit: Same as input
  Out1 : Outport  VectorParamsAs1DForOutWhenUnconnected=off
  wires:
  DummyGain/1 -> Out1/1
  In1/1 -> DummyGain/1

== system ASM_Traffic_new/Environment/Interface_Out/Plant_ModelSignals/a_x_Min[m|s2]_ ==
  In1 : Inport
  DummyGain : Gain  SaturateOnIntegerOverflow=on  OutDataTypeStr=Inherit: Same as input  ParamDataTypeStr=Inherit: Same as input
  Out1 : Outport  VectorParamsAs1DForOutWhenUnconnected=off
  wires:
  In1/1 -> DummyGain/1
  DummyGain/1 -> Out1/1

== system ASM_Traffic_new/Environment/Interface_Out/Plant_ModelSignals/a_x_Vehicle_Ref_TrafficDriver[m|s2]_ ==
  In1 : Inport
  Gain : Gain  SaturateOnIntegerOverflow=on  OutDataTypeStr=Inherit: Same as input  ParamDataTypeStr=Inherit: Same as input
  Out1 : Outport  VectorParamsAs1DForOutWhenUnconnected=off
  wires:
  Gain/1 -> Out1/1
  In1/1 -> Gain/1

== system ASM_Traffic_new/Environment/Interface_Out/Plant_ModelSignals/a_y_Max[m|s2]_ ==
  In1 : Inport
  DummyGain : Gain  SaturateOnIntegerOverflow=on  OutDataTypeStr=Inherit: Same as input  ParamDataTypeStr=Inherit: Same as input
  Out1 : Outport  VectorParamsAs1DForOutWhenUnconnected=off
  wires:
  DummyGain/1 -> Out1/1
  In1/1 -> DummyGain/1

== system ASM_Traffic_new/Environment/Interface_Out/Plant_ModelSignals/d_Total_Fellows[m]_ ==
  In1 : Inport
  Gain : Gain  SaturateOnIntegerOverflow=on  OutDataTypeStr=Inherit: Same as input  ParamDataTypeStr=Inherit: Same as input
  Out1 : Outport  VectorParamsAs1DForOutWhenUnconnected=off
  wires:
  In1/1 -> Gain/1
  Gain/1 -> Out1/1

== system ASM_Traffic_new/Environment/Interface_Out/Plant_ModelSignals/d_Vehicle_Road[m]_ ==
  In1 : Inport
  Gain : Gain  SaturateOnIntegerOverflow=on  OutDataTypeStr=Inherit: Same as input  ParamDataTypeStr=Inherit: Same as input
  Out1 : Outport  VectorParamsAs1DForOutWhenUnconnected=off
  wires:
  In1/1 -> Gain/1
  Gain/1 -> Out1/1

== system ASM_Traffic_new/Environment/Interface_Out/Plant_ModelSignals/n_Engine_Set[rpm]_ ==
  In1 : Inport
  DummyGain : Gain  SaturateOnIntegerOverflow=on  OutDataTypeStr=Inherit: Same as input  ParamDataTypeStr=Inherit: Same as input
  Out1 : Outport  VectorParamsAs1DForOutWhenUnconnected=off
  wires:
  In1/1 -> DummyGain/1
  DummyGain/1 -> Out1/1

== system ASM_Traffic_new/Environment/Interface_Out/Plant_ModelSignals/p_Ambient[Pa]_ ==
  In1 : Inport
  Gain : Gain  SaturateOnIntegerOverflow=on  OutDataTypeStr=Inherit: Same as input  ParamDataTypeStr=Inherit: Same as input
  Out1 : Outport  VectorParamsAs1DForOutWhenUnconnected=off
  wires:
  In1/1 -> Gain/1
  Gain/1 -> Out1/1

== system ASM_Traffic_new/Environment/Interface_Out/Plant_ModelSignals/q_dt_Vehicle_Init[6x1]_ ==
  In1 : Inport
  Gain : Gain  SaturateOnIntegerOverflow=on  OutDataTypeStr=Inherit: Same as input  ParamDataTypeStr=Inherit: Same as input
  Out1 : Outport  VectorParamsAs1DForOutWhenUnconnected=off
  wires:
  In1/1 -> Gain/1
  Gain/1 -> Out1/1

== system ASM_Traffic_new/Environment/Interface_Out/Plant_ModelSignals/s_Fellows_Ref[m]_ ==
  In1 : Inport
  Gain : Gain  SaturateOnIntegerOverflow=on  OutDataTypeStr=Inherit: Same as input  ParamDataTypeStr=Inherit: Same as input
  Out1 : Outport  VectorParamsAs1DForOutWhenUnconnected=off
  wires:
  In1/1 -> Gain/1
  Gain/1 -> Out1/1

== system ASM_Traffic_new/Environment/Interface_Out/Plant_ModelSignals/s_Total_Vehicle_Road[m]_ ==
  In1 : Inport
  Gain : Gain  SaturateOnIntegerOverflow=on  OutDataTypeStr=Inherit: Same as input  ParamDataTypeStr=Inherit: Same as input
  Out1 : Outport  VectorParamsAs1DForOutWhenUnconnected=off
  wires:
  Gain/1 -> Out1/1
  In1/1 -> Gain/1

== system ASM_Traffic_new/Environment/Interface_Out/Plant_ModelSignals/s_Vehicle_Init[m]_ ==
  In1 : Inport
  Gain : Gain  SaturateOnIntegerOverflow=on  OutDataTypeStr=Inherit: Same as input  ParamDataTypeStr=Inherit: Same as input
  Out1 : Outport  VectorParamsAs1DForOutWhenUnconnected=off
  wires:
  Gain/1 -> Out1/1
  In1/1 -> Gain/1

== system ASM_Traffic_new/Environment/Interface_Out/Plant_ModelSignals/s_Vehicle_Road[m]_ ==
  In1 : Inport
  Gain : Gain  SaturateOnIntegerOverflow=on  OutDataTypeStr=Inherit: Same as input  ParamDataTypeStr=Inherit: Same as input
  Out1 : Outport  VectorParamsAs1DForOutWhenUnconnected=off
  wires:
  In1/1 -> Gain/1
  Gain/1 -> Out1/1

== system ASM_Traffic_new/Environment/Interface_Out/Plant_ModelSignals/v_Rel_Fellows[m|s]_ ==
  In1 : Inport
  Gain : Gain  SaturateOnIntegerOverflow=on  OutDataTypeStr=Inherit: Same as input  ParamDataTypeStr=Inherit: Same as input
  Out1 : Outport  VectorParamsAs1DForOutWhenUnconnected=off
  wires:
  In1/1 -> Gain/1
  Gain/1 -> Out1/1

== system ASM_Traffic_new/Environment/Interface_Out/Plant_ModelSignals/v_Vehicle_Preview_Ref_Maneuver[m|s]_ ==
  In1 : Inport
  DummyGain : Gain  SaturateOnIntegerOverflow=on  OutDataTypeStr=Inherit: Same as input  ParamDataTypeStr=Inherit: Same as input
  Out1 : Outport  VectorParamsAs1DForOutWhenUnconnected=off
  wires:
  In1/1 -> DummyGain/1
  DummyGain/1 -> Out1/1

== system ASM_Traffic_new/Environment/Interface_Out/Plant_ModelSignals/v_Vehicle_Ref_Maneuver[km|h]_ ==
  In1 : Inport
  DummyGain : Gain  SaturateOnIntegerOverflow=on  OutDataTypeStr=Inherit: Same as input  ParamDataTypeStr=Inherit: Same as input
  Out1 : Outport  VectorParamsAs1DForOutWhenUnconnected=off
  wires:
  DummyGain/1 -> Out1/1
  In1/1 -> DummyGain/1

== system ASM_Traffic_new/Environment/Interface_Out/Plant_ModelSignals/v_Wind_Coor_Sys_E[x;y;z][m|s]_ ==
  In1 : Inport
  Gain : Gain  SaturateOnIntegerOverflow=on  OutDataTypeStr=Inherit: Same as input  ParamDataTypeStr=Inherit: Same as input
  Out1 : Outport  VectorParamsAs1DForOutWhenUnconnected=off
  wires:
  In1/1 -> Gain/1
  Gain/1 -> Out1/1

== system ASM_Traffic_new/Environment/Interface_Out/Plant_ModelSignals/x_Preview_DriverCurv[m]_ ==
  In1 : Inport
  Gain : Gain  SaturateOnIntegerOverflow=on  OutDataTypeStr=Inherit: Same as input  ParamDataTypeStr=Inherit: Same as input
  Out1 : Outport  VectorParamsAs1DForOutWhenUnconnected=off
  wires:
  In1/1 -> Gain/1
  Gain/1 -> Out1/1

== system ASM_Traffic_new/Environment/Interface_Out/Plant_ModelSignals/y_Preview_DriverCurv[m]_ ==
  In1 : Inport
  Gain : Gain  SaturateOnIntegerOverflow=on  OutDataTypeStr=Inherit: Same as input  ParamDataTypeStr=Inherit: Same as input
  Out1 : Outport  VectorParamsAs1DForOutWhenUnconnected=off
  wires:
  Gain/1 -> Out1/1
  In1/1 -> Gain/1

== system ASM_Traffic_new/Environment/Maneuver/PlantModel/ASMSignalCollector ==
  UserInterface : Inport
  VehicleInitStates : Inport  Port=2
  ModeSignals : Inport  Port=3
  RefSignals : Inport  Port=4
  Bus Creator : BusCreator  Inputs=7
  Bus Selector8 : BusSelector  OutputSignals=ManualControl.Testbench,ManualControl.ParkingBrake,ManualControl.StartButton,ManualControl.AutomaticTransmission.Sw_TipShift[-1Down|0Off|1Up]
  Replace_ModeSignals : BusAssignment  AssignedSignals=ModeSignals,RefSignals
  Maneuver_Signals : Outport  VectorParamsAs1DForOutWhenUnconnected=off
  wires:
  VehicleInitStates/1 -> Bus Creator/3
  Bus Selector8/1 -> Bus Creator/4  "<Testbench>"
  Bus Creator/1 -> Maneuver_Signals/1  "Maneuver"
  [ASMBUS_Environment_Mnvr_UserSignalsCustomized] -> Bus Creator/2
  [ASMBUS_Environment_ManeuverScheduler] -> Replace_ModeSignals/1
  Bus Selector8/2 -> Bus Creator/5  "<ParkingBrake>"
  Bus Selector8/3 -> Bus Creator/6  "<StartButton>"
  Bus Selector8/4 -> Bus Creator/7  "<Sw_TipShift[-1Down|0Off|1Up]>"
  ModeSignals/1 -> Replace_ModeSignals/2
  RefSignals/1 -> Replace_ModeSignals/3
  Replace_ModeSignals/1 -> Bus Creator/1  "ManeuverScheduler"
  UserInterface/1 -> Bus Selector8/1

== system ASM_Traffic_new/Environment/Maneuver/PlantModel/Customize_UserSignals ==
  UserSignals_In : Inport
  Bus Creator : BusCreator  Inputs=14
  Bus Selector1 : BusSelector  OutputSignals=User1[],User2[],User3[],User4[],User5[],User6[],User7[],User8[],User9[],User10[],User11[],User12[],User13[],User14[]
  CustomizedUserSignals : Subsystem
  ASMSignalBus : Outport  VectorParamsAs1DForOutWhenUnconnected=off
  UserSignals_Customized : Outport  Port=2  VectorParamsAs1DForOutWhenUnconnected=off
  wires:
  CustomizedUserSignals/8(Mnv_DataStream_8[]) -> Bus Creator/8
  CustomizedUserSignals/7(Mnv_DataStream_7[]) -> Bus Creator/7
  CustomizedUserSignals/6(Mnv_DataStream_6[]) -> Bus Creator/6
  CustomizedUserSignals/5(Mnv_DataStream_5[]) -> Bus Creator/5
  Bus Selector1/8 -> CustomizedUserSignals/8(User8[])  "<User8[]>"
  Bus Selector1/7 -> CustomizedUserSignals/7(User7[])  "<User7[]>"
  Bus Selector1/6 -> CustomizedUserSignals/6(User6[])  "<User6[]>"
  Bus Selector1/5 -> CustomizedUserSignals/5(User5[])  "<User5[]>"
  Bus Selector1/4 -> CustomizedUserSignals/4(User4[])  "<User4[]>"
  Bus Selector1/3 -> CustomizedUserSignals/3(User3[])  "<User3[]>"
  CustomizedUserSignals/3(ASM_Vehicle_TurnLights[]) -> Bus Creator/3
  CustomizedUserSignals/4(ECU_Commands[]) -> Bus Creator/4
  UserSignals_In/1 -> Bus Selector1/1
  Bus Creator/1 -> ASMSignalBus/1, UserSignals_Customized/1  "UserSignals_Customized"
  Bus Selector1/1 -> CustomizedUserSignals/1(User1[])  "<User1[]>"
  Bus Selector1/2 -> CustomizedUserSignals/2(User2[])  "<User2[]>"
  CustomizedUserSignals/1(ExternalSegmentEnd_Mode[]) -> Bus Creator/1
  CustomizedUserSignals/2(ExternalSegmentEnd_Value[]) -> Bus Creator/2
  Bus Selector1/9 -> CustomizedUserSignals/9(User9[])  "<User9[]>"
  Bus Selector1/10 -> CustomizedUserSignals/10(User10[])  "<User10[]>"
  Bus Selector1/11 -> CustomizedUserSignals/11(User11[])  "<User11[]>"
  Bus Selector1/12 -> CustomizedUserSignals/12(User12[])  "<User12[]>"
  Bus Selector1/13 -> CustomizedUserSignals/13(User13[])  "<User13[]>"
  Bus Selector1/14 -> CustomizedUserSignals/14(User14[])  "<User14[]>"
  CustomizedUserSignals/9(Mnv_DoorFL[]) -> Bus Creator/9
  CustomizedUserSignals/10(Mnv_DoorFR[]) -> Bus Creator/10
  CustomizedUserSignals/11(Mnv_DoorRL[]) -> Bus Creator/11
  CustomizedUserSignals/12(Mnv_DoorRR[]) -> Bus Creator/12
  CustomizedUserSignals/13(Mnv_Hood[]) -> Bus Creator/13
  CustomizedUserSignals/14(Mnv_Trunk[]) -> Bus Creator/14

== system ASM_Traffic_new/Environment/Maneuver/PlantModel/ExternalSegmentEnd ==
  In : Inport
  UserSignals_Customized : Inport  Port=2
  AvoidAlgLoop{1..9} (9 alike) : UnitDelay  SampleTime=-1  HasFrameUpgradeWarning=on
  Bus Selector : BusSelector  OutputSignals=ExternalSegmentEnd_Mode[],ExternalSegmentEnd_Value[]
  Bus Selector1 : BusSelector  OutputSignals=Plant.Traffic_Signals_toEnvironment.UserSignals_Customized.ManeuverSegmentEndTrigger[0|1]
  Bus Selector2 : BusSelector  OutputSignals=Plant.Road_ASMVeh.s_Veh_Road[m]
  Bus Selector3 : BusSelector  OutputSignals=Road,Interface_In,Sensors,Traffic
  Bus Selector4 : BusSelector  OutputSignals=ExternalModel.RollRate_Vehicle_CoG[deg|s]
  Bus Selector5 : BusSelector  OutputSignals=Plant.Object_Sensor_3D.Sensor_1_Front_Long,Plant.Object_Sensor_3D.Sensor_3_Rear
  Bus Selector6 : BusSelector  OutputSignals=ExternalModel.AEB[0|1],ExternalModel.FCW[0|1]
  Bus Selector7 : BusSelector  OutputSignals=SensorOutput.Dist_Object[m]
  Bus Selector8 : BusSelector  OutputSignals=SensorOutput.Dist_Object[m]
  Const_External_SegmentEnd_10[0|1] : Constant  Value=0
  Const_External_SegmentEnd_11_25 : Constant  Value=zeros(15,1)
  Const_External_SegmentEnd_5[0|1] : Constant  Value=0
  Const_External_SegmentEnd_6[0|1] : Constant  Value=0
  Const_External_SegmentEnd_7[0|1] : Constant  Value=0
  Const_External_SegmentEnd_8[0|1] : Constant  Value=0
  Const_External_SegmentEnd_9[0|1] : Constant  Value=0
  Dist_Front_Min : Subsystem
  Dist_Rear_Min : Subsystem
  Mux : Mux  Inputs=[1 1 1 1 1 1 1 1 1 1 15]
  SegmentEndTrigger : Subsystem
  External_SegmentEnd[0|1] : Outport  VectorParamsAs1DForOutWhenUnconnected=off
  wires:
  Bus Selector7/1 -> Dist_Front_Min/1(Dist_Front[m])  "<Dist_Object[m]>"
  AvoidAlgLoop9/1 -> Mux/4
  AvoidAlgLoop8/1 -> Mux/3
  Bus Selector6/2 -> AvoidAlgLoop9/1  "<FCW[0|1]>"
  Bus Selector6/1 -> AvoidAlgLoop8/1  "<AEB[0|1]>"
  Const_External_SegmentEnd_5[0|1]/1 -> Mux/5
  Const_External_SegmentEnd_6[0|1]/1 -> Mux/6
  Const_External_SegmentEnd_7[0|1]/1 -> Mux/7
  Const_External_SegmentEnd_8[0|1]/1 -> Mux/8
  Const_External_SegmentEnd_9[0|1]/1 -> Mux/9
  Const_External_SegmentEnd_10[0|1]/1 -> Mux/10
  Mux/1 -> External_SegmentEnd[0|1]/1
  Bus Selector3/4 -> Bus Selector1/1  "<Traffic>"
  Bus Selector1/1 -> AvoidAlgLoop6/1  "<ManeuverSegmentEndTrigger[0|1]>"
  AvoidAlgLoop6/1 -> Mux/2
  UserSignals_Customized/1 -> Bus Selector/1
  Bus Selector/1 -> AvoidAlgLoop1/1  "<ExternalSegmentEnd_Mode[]>"
  Bus Selector/2 -> AvoidAlgLoop2/1  "<ExternalSegmentEnd_Value[]>"
  Bus Selector3/2 -> Bus Selector6/1, Bus Selector4/1  "<Interface_In>"
  Bus Selector4/1 -> AvoidAlgLoop4/1  "<RollRate_Vehicle_CoG[deg|s]>"
  Bus Selector2/1 -> AvoidAlgLoop3/1  "<s_Veh_Road[m]>"
  AvoidAlgLoop1/1 -> SegmentEndTrigger/1(ExternalSegmentEnd_Mode[])
  AvoidAlgLoop2/1 -> SegmentEndTrigger/2(ExternalSegmentEnd_Value[])
  AvoidAlgLoop3/1 -> SegmentEndTrigger/3(s_Road[m])
  AvoidAlgLoop4/1 -> SegmentEndTrigger/4(RollRate_Vehicle[deg|s])
  Dist_Front_Min/1(Out1) -> AvoidAlgLoop5/1
  Dist_Rear_Min/1(Out1) -> AvoidAlgLoop7/1
  AvoidAlgLoop7/1 -> SegmentEndTrigger/6(Distance_Rear[m])
  AvoidAlgLoop5/1 -> SegmentEndTrigger/5(Distance_Front[m])
  SegmentEndTrigger/1(External_SegmentEnd[0|1]) -> Mux/1
  Const_External_SegmentEnd_11_25/1 -> Mux/11
  In/1 -> Bus Selector3/1
  Bus Selector3/1 -> Bus Selector2/1  "<Road>"
  Bus Selector3/3 -> Bus Selector5/1  "<Sensors>"
  Bus Selector5/1 -> Bus Selector7/1  "<Sensor_1_Front_Long>"
  Bus Selector5/2 -> Bus Selector8/1  "<Sensor_3_Rear>"
  Bus Selector8/1 -> Dist_Rear_Min/1(Dist_Rear[m])  "<Dist_Object[m]>"

== system ASM_Traffic_new/Environment/Maneuver/PlantModel/ExternalUserData ==
  Angle_SteeringWheel[deg] : Constant  Value=0
  Bus Creator2 : BusCreator  Inputs=10
  Gear[] : Constant  Value=0
  LaneIdx_Ref[] : Constant  Value=0
  Pos_AccPedal[%] : Constant  Value=0
  Pos_BrakePedal[%] : Constant  Value=0
  Pos_ClutchPedal[%] : Constant  Value=100
  "SelectorLever[] " : Constant  Value=0
  Trq_Steering[Nm] : Constant  Value=0
  d_Ref[m] : Constant  Value=0
  v_Vehicle_Ref[m|s] : Constant  Value=0
  External_ReferenceSignals : Outport  VectorParamsAs1DForOutWhenUnconnected=off
  wires:
  "SelectorLever[] "/1 -> Bus Creator2/10  "SelectorLever[]"
  Trq_Steering[Nm]/1 -> Bus Creator2/9  "Trq_Steering[Nm]"
  Angle_SteeringWheel[deg]/1 -> Bus Creator2/5  "Angle_SteeringWheel[deg]"
  Gear[]/1 -> Bus Creator2/4  "Gear[]"
  Pos_ClutchPedal[%]/1 -> Bus Creator2/3  "Pos_ClutchPedal[%]"
  Pos_BrakePedal[%]/1 -> Bus Creator2/2  "Pos_BrakePedal[%]"
  Pos_AccPedal[%]/1 -> Bus Creator2/1  "Pos_AccPedal[%]"
  v_Vehicle_Ref[m|s]/1 -> Bus Creator2/6  "v_Vehicle_Ref[m|s]"
  d_Ref[m]/1 -> Bus Creator2/7  "d_Ref[m]"
  LaneIdx_Ref[]/1 -> Bus Creator2/8  "LaneIdx_Ref[]"
  Bus Creator2/1 -> External_ReferenceSignals/1
